simulink model "sfRobotExample"  (R2025b)
settings: Solver=VariableStepAuto  StartTime=0.0  StopTime=inf  RelTol=1e-3
PreLoadFcn:
  | tMax = 250;
  | dock = [8 5];
  | dockWidth = 0.25;
  | circles = [3 8 1; 8 2 1; 13 8 1];
  | boxes = [2 3.5 2 3; 6 9 4 2; 12 3.5 2 3];
StopFcn:
  | hold off
libraries: sfRobotExampleLib x4
settings Model: Creator=The MathWorks, Inc.  LastModifiedBy=The MathWorks, Inc.
settings SolverCC: MaxZcPerStep=1.0
settings OptimizationCC: ReuseModelBlockBuffer=off
settings DebuggingCC: UnconnectedInputMsg=warning  UnconnectedOutputMsg=warning  UnconnectedLineMsg=warning
settings ModelReferenceCC: EnableRefExpFcnMdlSchedulingChecks=on
settings RTWCC: GPUComputeCapability=3.5  DLArmComputeVersion=19.05

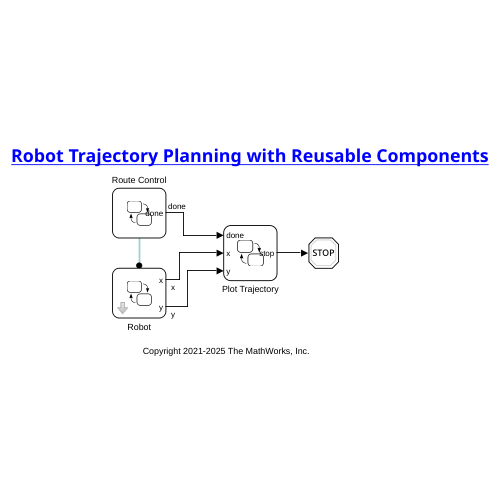
[thumbnail: Simulink's stored preview of the top-level diagram]
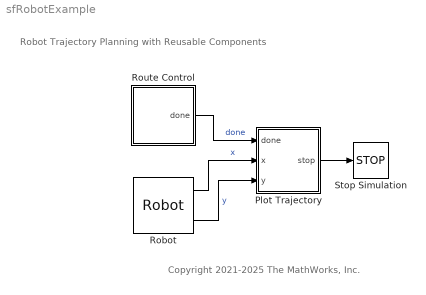
== system sfRobotExample ==
  note: Copyright 2021-2025 The MathWorks, Inc.
  note: Robot Trajectory Planning with Reusable Components
  Plot Trajectory : Stateflow chart  TreatAsAtomicUnit=on
      settings: PortSchema="{\"entries\":[{\"content\":{\"sides\":[{\"content\":{\"connectorIds\":[\"In3\",\"In1\",\"In2\"]},\"type\":\"ConnectorPlacement.EquallySpacedRectSide\",\"uuid\":\"e16a7123-7319-4739-8098-e155df048508\"},{\"content\":{\"connectorIds\":[\"Out1\"],\"side\":\"RIGHT\"},\"type\":\"ConnectorPlacement.EquallySpacedRectSide\",\"uuid\":\"31f7066e-6ef4-4e57-a064-0190e66f0086\"},{\"content\":{\"connectorIds\":[],\"side\":\"TOP\"},\"type\":\"ConnectorPlacement.EquallySpacedRectSide\",\"uuid\":\"619d4e31-97a3-4d20-aef7-7a441a173d24\"}]},\"type\":\"ConnectorPlacement.EquallySpacedConnector\",\"uuid\":\"7c1589f4-674e-4c3e-befb-66868fbf03bf\"}],\"packageUris\":[\"http://schema.mathworks.com/mf0/Connector/R2020b\"],\"version\":\"1.0\"}"
  Robot : sfRobotExampleLib/Robot  startPos=[0 0]  startDir=3
  Route Control : Stateflow chart  TreatAsAtomicUnit=on
  Stop Simulation : Stop
  wires:
  Robot/2 -> Plot Trajectory/2(y)  "y"
  Robot/1 -> Plot Trajectory/1(x)  "x"
  Route Control/1(done) -> Plot Trajectory/3(done)  "done"
  Plot Trajectory/1(stop) -> Stop Simulation/1

== stateflow chart sfRobotExample/Plot Trajectory ==
  state Init
    coder.extrinsic('sfRobotScene','plot','hold');
    sfRobotScene(dock,dockWidth,boxes,circles);
    xPrev = x;
    yPrev = y;
  state Plot
    plot([xPrev,x],[yPrev,y],'ob');
    xPrev = x;
    yPrev = y;
  state End
    plot([xPrev,x],[yPrev,y],'ob');
    stop = true;
  (default) -> Init
  Init -> Plot
  Plot -> End : [done]
  data: dock parameter double size=[1 2]; boxes parameter; circles parameter; xPrev local double size=1; yPrev local double size=1; x input; y input; done input boolean size=1; stop output boolean =false; dockWidth parameter double size=1

== stateflow chart sfRobotExample/Route Control ==
  state Run
    state Move
    state ContactDock
    state Rotate
    (default) -> Move : {speed = 0.5;}
    24 -> (junction 52)
    (junction 44) -> Move
    (junction 81) -> (junction 44)
    (junction 52) -> (junction 50)
    (junction 38) -> (junction 44) [order 2]
    (junction 79) -> (junction 81) : {speed = 0.1;}
    23 -> ContactDock
    100 -> (junction 38)
    (junction 38) -> (junction 79) [order 1] : [distToDock < 2]
    (junction 41) -> (junction 38)
    101 -> 70
    (junction 50) -> 69
    71 -> (junction 41)
  state Stop
    done = true;
  (default) -> Run
  Run -> Stop [order 1] : [distToDock<dockWidth]
  Run -> Stop [order 2] : after(tMax,sec)
      | {coder.extrinsic('warning');
      | warning('Unable to reach dock.');}
  data: speed function_input; distToDock function_output; distToDock local double size=1 =Inf; speed local double size=1; tMax parameter; done output boolean size=1 =false; dockWidth parameter
